simulink model "export_lab3"  (R2024b)
settings: Solver=FixedStepAuto  StartTime=0.0  StopTime=inf  FixedStep=0.02  MaxStep=0.1  RelTol=1e-3  EnableMultiTasking=on
PreLoadFcn:
  | % load parameters of the default quadrotor
  | disp('Quadrotor parameters loaded by PreLoadFcn')
  | mdl_quadrotor
undefined symbols (not defined in the file or in its folder): Angular, Linear, rot2
libraries: robotlib x3
settings Model: Creator=corkep  LastModifiedBy=david
settings SolverCC: AlgebraicLoopSolver=TrustRegion
settings DataIOCC: LimitDataPoints=on  ReturnWorkspaceOutputs=off
settings OptimizationCC: ReuseModelBlockBuffer=off  ExpressionDepthLimit=2147483647  LifeSpan=inf
settings DebuggingCC: UnderspecifiedInitializationDetection=Classic  MergeDetectMultiDrivingBlocksExec=none  SolverPrmCheckMsg=warning  UnconnectedInputMsg=warning  UnconnectedOutputMsg=warning  UnconnectedLineMsg=warning  AllowSymbolicDim=off  StateNameClashWarn=warning  SFUnexpectedBacktrackingDiag=warning  SFNoUnconditionalDefaultTransitionDiag=warning  SFExecutionAtInitializationDiag=none  ArithmeticOperatorsInVariantConditions=warning
settings HardwareCC: ProdBitPerPointer=32  ProdBitPerSizeT=32  ProdBitPerPtrDiffT=32  ProdLargestAtomicFloat=None  ProdIntDivRoundTo=Undefined  ProdEndianess=Unspecified  ProdWordSize=32  ProdHWDeviceType=32-bit Generic
settings ModelReferenceCC: EnableRefExpFcnMdlSchedulingChecks=on  PropagateSignalLabelsOutOfModel=off
settings SFSimCC: SimUseLocalCustomCode=off  CustomCodeUndefinedFunction=UseInterfaceOnly
settings RTWCC: RTWUseLocalCustomCode=off  GPUComputeCapability=3.5  DLArmComputeVersion=19.05
settings CodeAppCC: StateflowObjectComments=on
settings GRTTargetCC: TargetLangStandard=C89/C90 (ANSI)  CombineOutputUpdateFcns=off  GRTInterface=on
settings ConfigComp: CovMetricSettings=dw  CovSaveCumulativeToWorkspaceVar=on  CovSaveSingleToWorkspaceVar=on  CovExternalEMLEnable=off  CovSFcnEnable=off  CovBoundaryAbsTol=1.0e-5

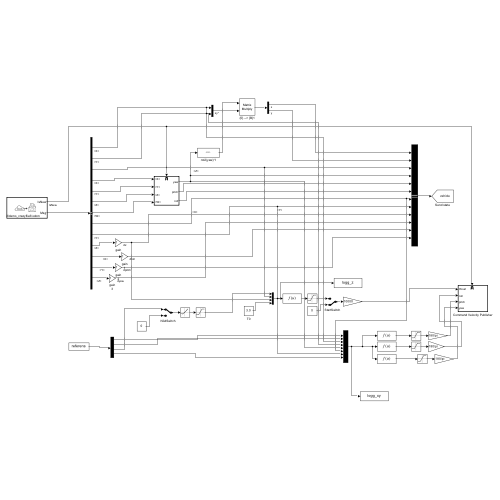
[thumbnail: Simulink's stored preview of the top-level diagram]
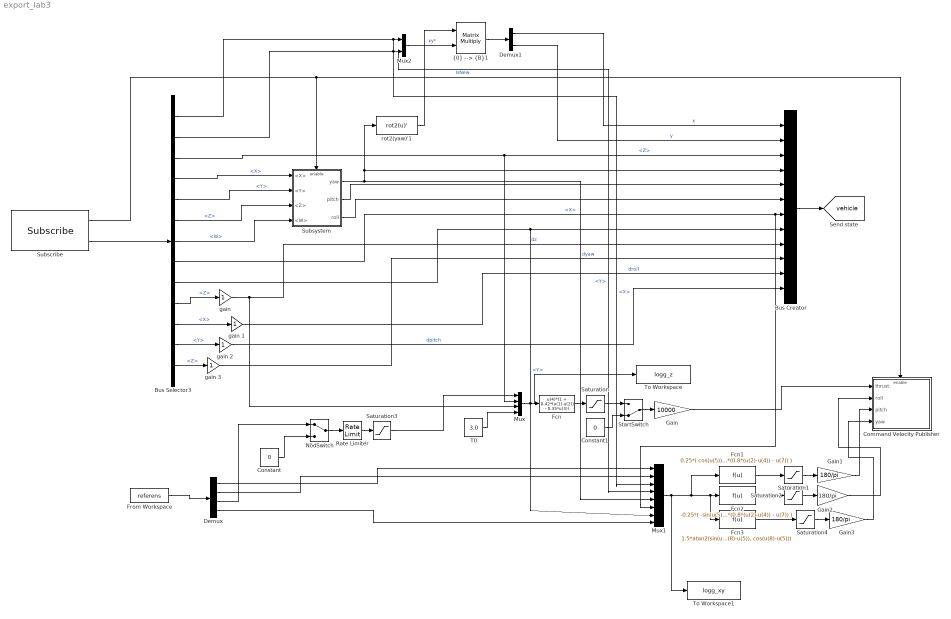
== system export_lab3 ==
  Bus Creator : BusCreator  Inputs=12
  Bus Selector3 : BusSelector  OutputSignals=Pose.Pose.Position.X,Pose.Pose.Position.Y,Pose.Pose.Position.Z,Pose.Pose.Orientation.X,Pose.Pose.Orientation.Y,Pose.Pose.Orientation.Z,Pose.Pose.Orientation.W,Twist.Twist.Linear.X,Twist.Twist.Linear.Y,Twist.Twist.Linear.Z,Twist.Twist.Angular.X,Twist.Twist.Angular.Y,Twist.Twist.Angular.Z
  Command Velocity Publisher : Subsystem
  Constant : Constant  Value=0
  Constant1 : Constant  Value=0
  Demux : Demux
  Demux1 : Demux  Outputs=2
  Fcn : Fcn  Expr=u(4)*(1 + 0.42*(u(1)-u(2)) - 0.35*u(3))
  Fcn1 : Fcn  Expr=0.25*( cos(u(5))*(0.8*(u(1)-u(3)) - u(6)) + sin(u(5))*(0.8*(u(2)-u(4)) - u(7)) )
  Fcn2 : Fcn  Expr=-0.25*( -sin(u(5))*(0.8*(u(1)-u(3)) - u(6)) + cos(u(5))*(0.8*(u(2)-u(4)) - u(7)) )
  Fcn3 : Fcn  Expr=1.5*atan2(sin(u(8)-u(5)), cos(u(8)-u(5)))
  From Workspace : FromWorkspace  VariableName=referens  OutputAfterFinalValue=Holding final value
  Gain : Gain  Gain=10000
  Gain1 : Gain  Gain=180/pi
  Gain2 : Gain  Gain=180/pi
  Gain3 : Gain  Gain=180/pi
  Mux : Mux
  Mux1 : Mux  Inputs=8
  Mux2 : Mux  Inputs=2
  NödSwitch : ManualSwitch
  Rate Limiter : RateLimiter  RisingSlewLimit=0.2  FallingSlewLimit=-0.2  SampleTimeMode=inherited
  Saturation : Saturate  UpperLimit=6  LowerLimit=0
  Saturation1 : Saturate  UpperLimit=0.15  LowerLimit=-0.15
  Saturation2 : Saturate  UpperLimit=0.15  LowerLimit=-0.15
  Saturation3 : Saturate  UpperLimit=1.8  LowerLimit=0
  Saturation4 : Saturate  UpperLimit=1  LowerLimit=-1
  StartSwitch : ManualSwitch  CurrentSetting=0
  Subscribe : robotlib/Subscribe  topicSource=Select from ROS network  topic=/pixy/vicon/demo_crazyflie3/demo_crazyflie3/odom  messageType=nav_msgs/Odometry  SampleTime=-1  legacyBusStruct=off  messageQueueLength=51
  Subsystem : Subsystem
  T0 : Constant  Value=3.0
  To Workspace : ToWorkspace  VariableName=logg_z  SaveFormat=Timeseries  SampleTime=-1
  To Workspace1 : ToWorkspace  VariableName=logg_xy  SaveFormat=Timeseries  SampleTime=-1
  gain {,1..3} (4 alike) : Gain
  rot2(yaw)'1 : MATLABFcn  MATLABFcn=rot2(u)'  OutputDimensions=[2 2]  Output1D=off
  "{0} --> {B}1" : Product  Multiplication=Matrix(*)  RndMeth=Zero
  tag scope: vehicle=global
  wires:
  Bus Selector3/11 -> gain 1/1  "<X>"
  Bus Selector3/13 -> gain 3/1  "<Z>"
  Bus Selector3/10 -> "gain "/1  "<Z>"
  Bus Selector3/9 -> Bus Creator/8, Mux1/7  "<Y>"
  Bus Selector3/8 -> Mux1/6, Bus Creator/7  "<X>"
  Bus Selector3/3 -> Bus Creator/3, Mux/2  "<Z>"
  Bus Creator/1 -> [vehicle]
  Bus Selector3/12 -> gain 2/1  "<Y>"
  Subscribe/2 -> Bus Selector3/1
  Subscribe/1 -> Subsystem/Enable, Command Velocity Publisher/Enable  "IsNew"
  Mux2/1 -> "{0} --> {B}1"/2  "xy*"
  "{0} --> {B}1"/1 -> Demux1/1
  Demux1/1 -> Bus Creator/1  "x"
  Demux1/2 -> Bus Creator/2  "y"
  Bus Selector3/1 -> Mux1/3, Mux2/1  "<X>"
  Bus Selector3/2 -> Mux1/4, Mux2/2  "<Y>"
  rot2(yaw)'1/1 -> "{0} --> {B}1"/1
  "gain "/1 -> Bus Creator/9, Mux/3  "dz"
  gain 1/1 -> Bus Creator/11  "droll"
  gain 2/1 -> Bus Creator/12  "dpitch"
  gain 3/1 -> Bus Creator/10  "dyaw"
  Subsystem/1(yaw) -> Mux1/5, rot2(yaw)'1/1, Bus Creator/4
  Bus Selector3/4 -> Subsystem/1(<X>)  "<X>"
  Bus Selector3/5 -> Subsystem/2(<Y>)  "<Y>"
  Bus Selector3/6 -> Subsystem/3(<Z>)  "<Z>"
  Bus Selector3/7 -> Subsystem/4(<W>)  "<W>"
  Subsystem/2(pitch) -> Bus Creator/5
  Subsystem/3(roll) -> Bus Creator/6
  Constant1/1 -> StartSwitch/2
  NödSwitch/1 -> Rate Limiter/1
  StartSwitch/1 -> Gain/1
  Saturation3/1 -> Mux/1
  T0/1 -> Mux/4
  Rate Limiter/1 -> Saturation3/1
  Constant/1 -> NödSwitch/2
  Demux/3 -> NödSwitch/1
  Mux/1 -> To Workspace/1, Fcn/1
  Gain/1 -> Command Velocity Publisher/1(thrust)
  Saturation/1 -> StartSwitch/1
  Fcn/1 -> Saturation/1
  Mux1/1 -> To Workspace1/1, Fcn3/1, Fcn2/1, Fcn1/1
  Fcn3/1 -> Saturation4/1
  Fcn2/1 -> Saturation2/1
  Fcn1/1 -> Saturation1/1
  Saturation1/1 -> Gain1/1
  Saturation2/1 -> Gain2/1
  Saturation4/1 -> Gain3/1
  Gain1/1 -> Command Velocity Publisher/3(pitch)
  Gain2/1 -> Command Velocity Publisher/2(roll)
  Gain3/1 -> Command Velocity Publisher/4(yaw)
  From Workspace/1 -> Demux/1
  Demux/1 -> Mux1/1
  Demux/2 -> Mux1/2
  Demux/4 -> Mux1/8

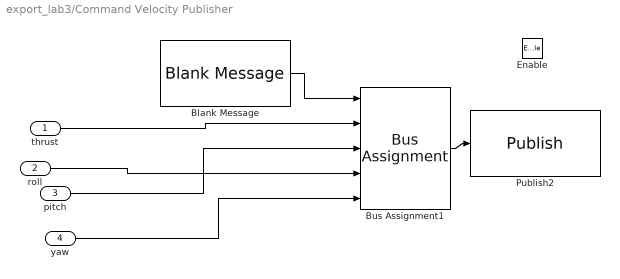
== system export_lab3/Command Velocity Publisher ==
  thrust : Inport
  roll : Inport  Port=2
  pitch : Inport  Port=3
  yaw : Inport  Port=4
  Enable : EnablePort
  Blank Message : robotlib/Blank Message  messageClass=Message  entityType=geometry_msgs/Twist  messageType=geometry_msgs/Twist  SampleTime=inf  legacyBusStruct=off
  Bus Assignment1 : BusAssignment  DialogController=Simulink.DDGSource_BusAssignment  AssignedSignals=Linear.Z,Linear.X,Linear.Y,Angular.Z
  Publish2 : robotlib/Publish  topicSource=Select from ROS network  topic=/demo_crazyflie3/cmd_vel  messageType=geometry_msgs/Twist  legacyBusStruct=off  messageQueueLength=105
  wires:
  Bus Assignment1/1 -> Publish2/1
  Blank Message/1 -> Bus Assignment1/1
  yaw/1 -> Bus Assignment1/5
  roll/1 -> Bus Assignment1/4
  pitch/1 -> Bus Assignment1/3
  thrust/1 -> Bus Assignment1/2

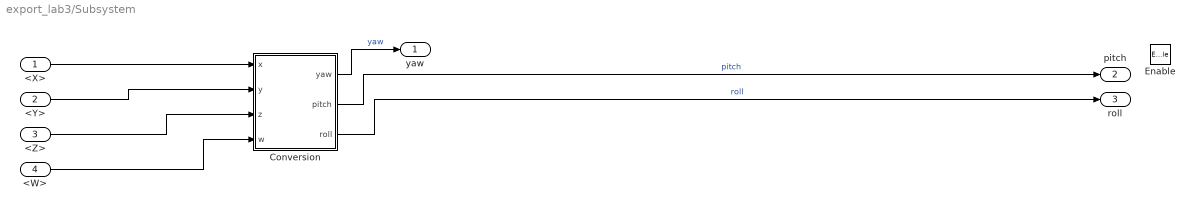
== system export_lab3/Subsystem ==
  <X> : Inport
  <Y> : Inport  Port=2
  <Z> : Inport  Port=3
  <W> : Inport  Port=4
  Enable : EnablePort
  Conversion : MATLAB Function  TreatAsAtomicUnit=on
  yaw : Outport
  pitch : Outport  Port=2
  roll : Outport  Port=3
  wires:
  Conversion/1(yaw) -> yaw/1  "yaw"
  <X>/1 -> Conversion/1(x)
  Conversion/2(pitch) -> pitch/1  "pitch"
  <W>/1 -> Conversion/4(w)
  <Y>/1 -> Conversion/2(y)
  Conversion/3(roll) -> roll/1  "roll"
  <Z>/1 -> Conversion/3(z)

== matlab function export_lab3/Subsystem/Conversion ==
  data: yaw output; x input; y input; z input; w input; pitch output; roll output
function [yaw,pitch,roll]  = quat2eul(x,y,z,w)
%#codegen

% Convert the quaternion to a yaw angle (zyx euler angle)
eul = quat2eul([w,x,y,z]);
yaw = eul(1);
roll = eul(3);
pitch = eul(2);

end
